simulink model "demo_ident"  (R2024b)
settings: Solver=ode3  StartTime=0.0  StopTime=max(time)  FixedStep=T_sample  RelTol=1e-3  EnableMultiTasking=on
values from neighbouring files (symbols this model uses):
  eta_i = x(3)    [LS_demo_ident.m]
  J = x(4)    [LS_demo_ident.m]
  K1 = x(1)    [LS_demo_ident.m]
  K2 = x(2)    [LS_demo_ident.m]
settings Model: Creator=shaocan  LastModifiedBy=sk3547969879
settings SolverCC: AlgebraicLoopSolver=TrustRegion
settings DataIOCC: LimitDataPoints=on  SaveFormat=Array  ReturnWorkspaceOutputs=off
settings OptimizationCC: LifeSpan=inf
settings DebuggingCC: UnconnectedInputMsg=warning  UnconnectedOutputMsg=warning  UnconnectedLineMsg=warning  SFUnexpectedBacktrackingDiag=warning  SFNoUnconditionalDefaultTransitionDiag=warning  SFExecutionAtInitializationDiag=none  ArithmeticOperatorsInVariantConditions=warning
settings HardwareCC: ProdBitPerPointer=32  ProdBitPerSizeT=32  ProdBitPerPtrDiffT=32  ProdLargestAtomicFloat=None  ProdIntDivRoundTo=Undefined  ProdEndianess=Unspecified  ProdWordSize=32  ProdHWDeviceType=32-bit Generic
settings ModelReferenceCC: EnableRefExpFcnMdlSchedulingChecks=on  PropagateSignalLabelsOutOfModel=off
settings SFSimCC: SimUseLocalCustomCode=off  CustomCodeUndefinedFunction=UseInterfaceOnly
settings RTWCC: RTWUseLocalCustomCode=off  GPUComputeCapability=3.5  DLArmComputeVersion=19.05
settings CodeAppCC: StateflowObjectComments=on
settings GRTTargetCC: TargetLangStandard=C89/C90 (ANSI)
settings ConfigComp: CovMetricSettings=dw  CovSaveCumulativeToWorkspaceVar=on  CovSaveSingleToWorkspaceVar=on  CovExternalEMLEnable=off  CovSFcnEnable=off

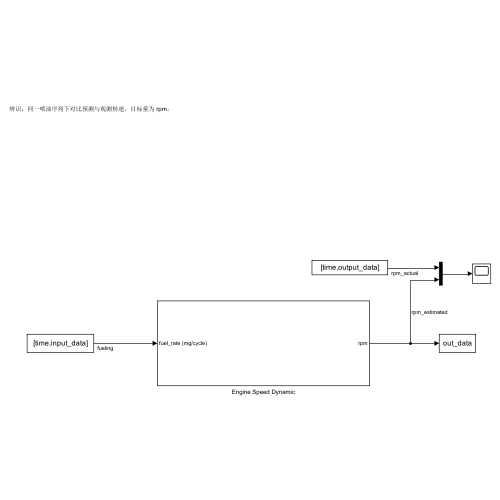
[thumbnail: Simulink's stored preview of the top-level diagram]
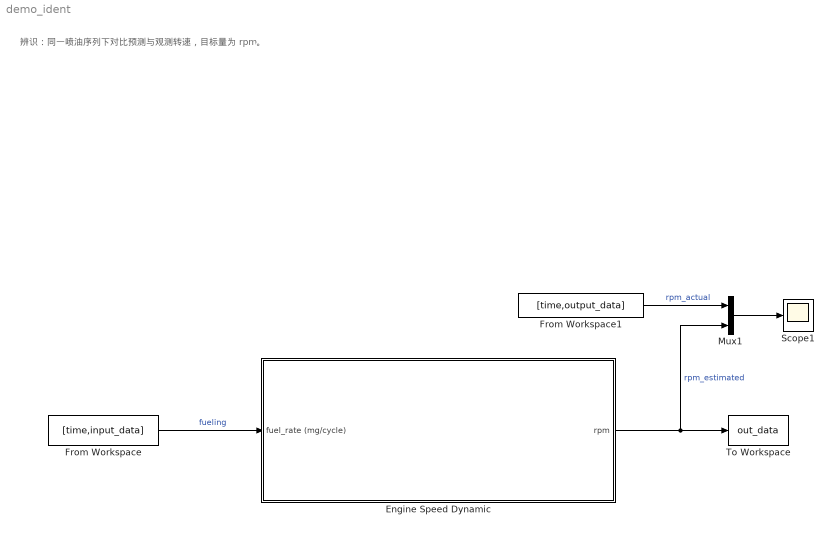
== system demo_ident ==
  note: 辨识：同一喷油序列下对比预测与观测转速，目标量为 rpm。
  Engine Speed Dynamic : Subsystem
  From Workspace : FromWorkspace  VariableName=[time,input_data]
  From Workspace1 : FromWorkspace  VariableName=[time,output_data]
  Mux1 : Mux  Inputs=2
  Scope1 : Scope
  To Workspace : ToWorkspace  VariableName=out_data  SaveFormat=Timeseries  SampleTime=-1
  wires:
  Mux1/1 -> Scope1/1
  Engine Speed Dynamic/1(rpm) -> To Workspace/1, Mux1/2  "rpm_estimated"
  From Workspace1/1 -> Mux1/1  "rpm_actual"
  From Workspace/1 -> Engine Speed Dynamic/1(fuel_rate (mg/cycle))  "fueling"

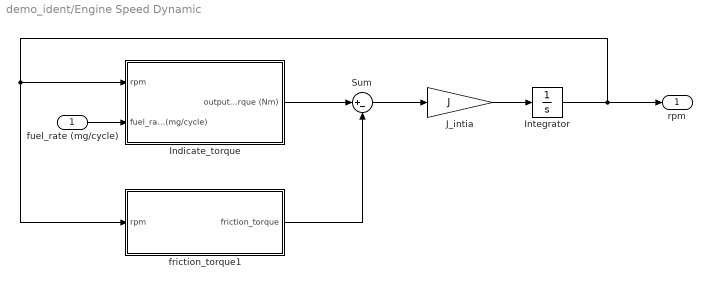
== system demo_ident/Engine Speed Dynamic ==
  fuel_rate (mg/cycle) : Inport
  Indicate_torque : Subsystem
  Integrator : Integrator  InitialCondition=960
  J_intia : Gain  Gain=J
  Sum : Sum  Inputs=|+-
  friction_torque1 : Subsystem
  rpm : Outport
  wires:
  Sum/1 -> J_intia/1
  Indicate_torque/1(output_torque (Nm)) -> Sum/1
  Integrator/1 -> rpm/1, friction_torque1/1(rpm), Indicate_torque/1(rpm)
  fuel_rate (mg/cycle)/1 -> Indicate_torque/2(fuel_rate (mg/cycle))
  friction_torque1/1(friction_torque) -> Sum/2
  J_intia/1 -> Integrator/1

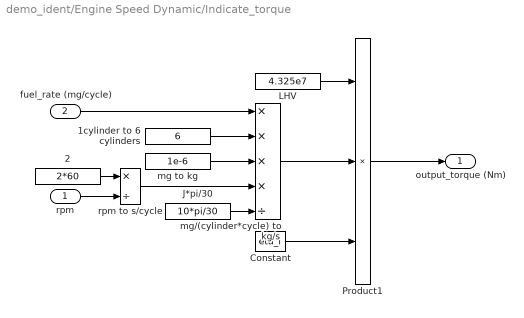
== system demo_ident/Engine Speed Dynamic/Indicate_torque ==
  rpm : Inport
  fuel_rate (mg/cycle) : Inport  Port=2
  1cylinder to 6 cylinders : Constant  Value=6
  2 : Constant  Value=2*60
  Constant : Constant  Value=eta_i
  J*pi/30 : Constant  Value=10*pi/30
  LHV : Constant  Value=4.325e7
  Product1 : Product  Inputs=3
  mg to kg : Constant  Value=1e-6
  mg/(cylinder*cycle) to kg/s : Product  Inputs=****/
  rpm to s/cycle : Product  Inputs=*/
  output_torque (Nm) : Outport
  wires:
  Product1/1 -> output_torque (Nm)/1
  Constant/1 -> Product1/3
  fuel_rate (mg/cycle)/1 -> mg/(cylinder*cycle) to kg/s/1
  1cylinder to 6 cylinders/1 -> mg/(cylinder*cycle) to kg/s/2
  2/1 -> rpm to s/cycle/1
  mg to kg/1 -> mg/(cylinder*cycle) to kg/s/3
  LHV/1 -> Product1/1
  J*pi/30/1 -> mg/(cylinder*cycle) to kg/s/5
  rpm to s/cycle/1 -> mg/(cylinder*cycle) to kg/s/4
  rpm/1 -> rpm to s/cycle/2
  mg/(cylinder*cycle) to kg/s/1 -> Product1/2

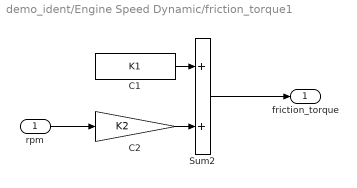
== system demo_ident/Engine Speed Dynamic/friction_torque1 ==
  rpm : Inport
  C1 : Constant  Value=K1
  C2 : Gain  Gain=K2
  Sum2 : Sum
  friction_torque : Outport
  wires:
  rpm/1 -> C2/1
  C1/1 -> Sum2/1
  C2/1 -> Sum2/2
  Sum2/1 -> friction_torque/1
